simulink subsystem "Controller"  (R2025b)
settings: Solver=VariableStepAuto  StartTime=0.0  StopTime=10.0  RelTol=1e-3
libraries: slpidlib x1
settings Model: Creator=Admin  LastModifiedBy=Admin

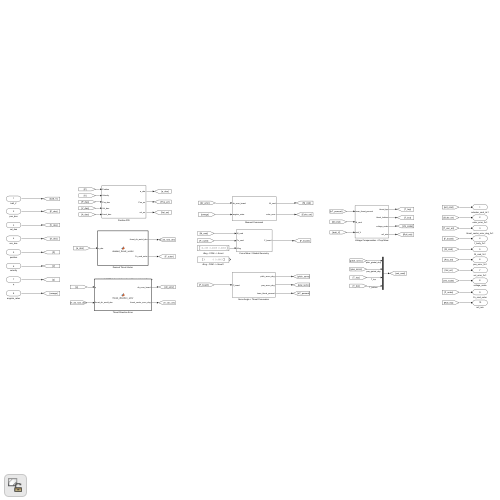
[thumbnail: Simulink's stored preview of the top-level diagram]
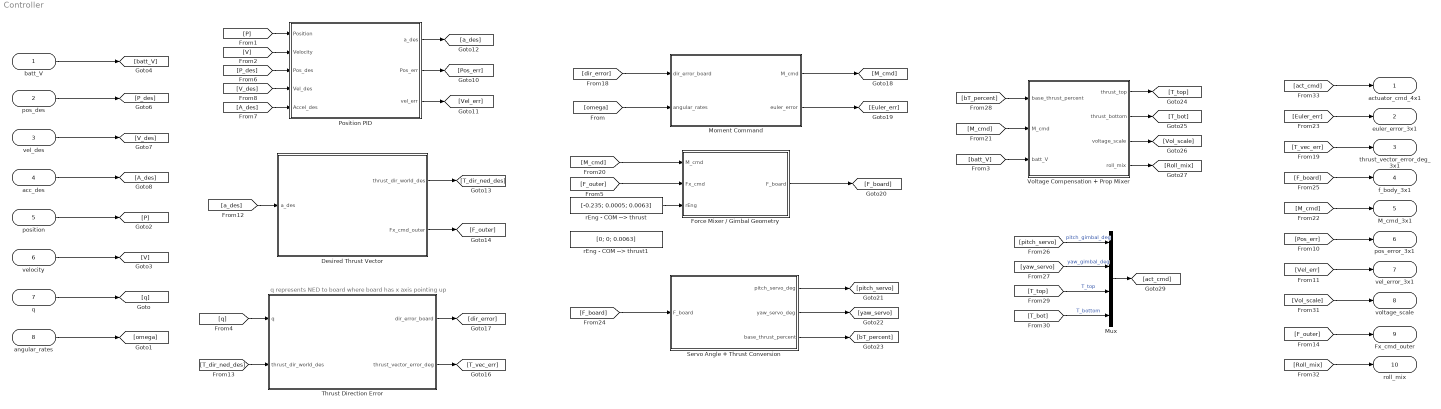
== system Controller ==
  note: q represents NED to board where board has x axis pointing up
  batt_V : Inport
  pos_des : Inport  Port=2
  vel_des : Inport  Port=3
  acc_des : Inport  Port=4
  position : Inport  Port=5
  velocity : Inport  Port=6
  q : Inport  Port=7
  angular_rates : Inport  Port=8
  Desired Thrust Vector : MATLAB Function  TreatAsAtomicUnit=on
  Force Mixer / Gimbal Geometry : Subsystem
  Moment Command : Subsystem
  Mux : Mux
  Position PID : Subsystem
  Servo Angle + Thrust Conversion : Subsystem
  Thrust Direction Error : MATLAB Function  TreatAsAtomicUnit=on
  Voltage Compensation + Prop Mixer : Subsystem
  rEng - COM --> thrust : Constant  Value=[-0.235; 0.0005; 0.0063]
  rEng - COM --> thrust1 : Constant  Value=[0; 0; 0.0063]
  actuator_cmd_4x1 : Outport
  euler_error_3x1 : Outport  Port=2
  thrust_vector_error_deg_3x1 : Outport  Port=3
  f_body_3x1 : Outport  Port=4
  M_cmd_3x1 : Outport  Port=5
  pos_error_3x1 : Outport  Port=6
  vel_error_3x1 : Outport  Port=7
  voltage_scale : Outport  Port=8
  Fx_cmd_outer : Outport  Port=9
  roll_mix : Outport  Port=10
  wires:
  [q] -> Thrust Direction Error/1(q)
  [omega] -> Moment Command/2(angular_rates)
  [P] -> Position PID/1(Position)
  [V] -> Position PID/2(Velocity)
  [P_des] -> Position PID/3(Pos_des)
  [A_des] -> Position PID/5(Accel_des)
  [V_des] -> Position PID/4(Vel_des)
  Position PID/2(Pos_err) -> [Pos_err]
  Position PID/3(vel_err) -> [Vel_err]
  [Pos_err] -> pos_error_3x1/1
  [Vel_err] -> vel_error_3x1/1
  [a_des] -> Desired Thrust Vector/1(a_des)
  Desired Thrust Vector/2(Fx_cmd_outer) -> [F_outer]
  [T_dir_ned_des] -> Thrust Direction Error/2(thrust_dir_world_des)
  [F_outer] -> Fx_cmd_outer/1
  [F_outer] -> Force Mixer / Gimbal Geometry/2(Fx_cmd)
  Thrust Direction Error/1(dir_error_board) -> [dir_error]
  Thrust Direction Error/2(thrust_vector_error_deg) -> [T_vec_err]
  [dir_error] -> Moment Command/1(dir_error_board)
  [T_vec_err] -> thrust_vector_error_deg_3x1/1
  Moment Command/1(M_cmd) -> [M_cmd]
  [M_cmd] -> Force Mixer / Gimbal Geometry/1(M_cmd)
  [M_cmd] -> M_cmd_3x1/1
  Moment Command/2(euler_error) -> [Euler_err]
  [Euler_err] -> euler_error_3x1/1
  Force Mixer / Gimbal Geometry/1(F_board) -> [F_board]
  [F_board] -> f_body_3x1/1
  Servo Angle + Thrust Conversion/1(pitch_servo_deg) -> [pitch_servo]
  Servo Angle + Thrust Conversion/2(yaw_servo_deg) -> [yaw_servo]
  Servo Angle + Thrust Conversion/3(base_thrust_percent) -> [bT_percent]
  [pitch_servo] -> Mux/1  "pitch_gimbal_deg"
  [yaw_servo] -> Mux/2  "yaw_gimbal_deg"
  [T_top] -> Mux/3  "T_top"
  [T_bot] -> Mux/4  "T_bottom"
  [Vol_scale] -> voltage_scale/1
  [Roll_mix] -> roll_mix/1
  Mux/1 -> [act_cmd]
  [act_cmd] -> actuator_cmd_4x1/1
  [bT_percent] -> Voltage Compensation + Prop Mixer/1(base_thrust_percent)
  [M_cmd] -> Voltage Compensation + Prop Mixer/2(M_cmd)
  [batt_V] -> Voltage Compensation + Prop Mixer/3(batt_V)
  Voltage Compensation + Prop Mixer/1(thrust_top) -> [T_top]
  Voltage Compensation + Prop Mixer/2(thrust_bottom) -> [T_bot]
  Voltage Compensation + Prop Mixer/3(voltage_scale) -> [Vol_scale]
  Voltage Compensation + Prop Mixer/4(roll_mix) -> [Roll_mix]
  Position PID/1(a_des) -> [a_des]
  Desired Thrust Vector/1(thrust_dir_world_des) -> [T_dir_ned_des]
  [F_board] -> Servo Angle + Thrust Conversion/1(F_board)
  batt_V/1 -> [batt_V]
  pos_des/1 -> [P_des]
  vel_des/1 -> [V_des]
  acc_des/1 -> [A_des]
  position/1 -> [P]
  velocity/1 -> [V]
  q/1 -> [q]
  angular_rates/1 -> [omega]
  rEng - COM --> thrust/1 -> Force Mixer / Gimbal Geometry/3(rEng)

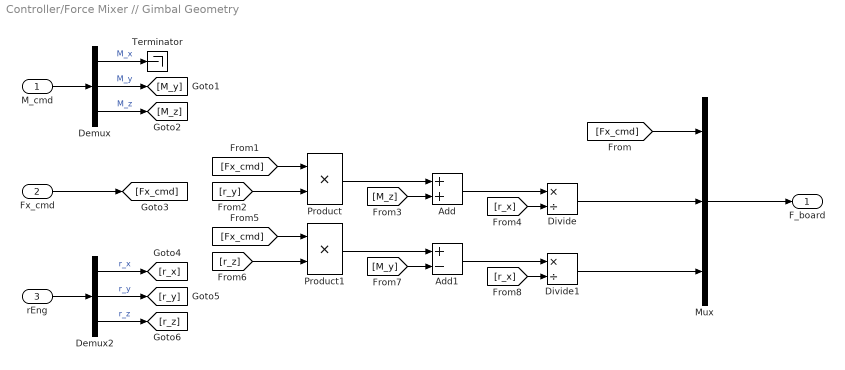
== system Controller/Force Mixer // Gimbal Geometry ==
  M_cmd : Inport
  Fx_cmd : Inport  Port=2
  rEng : Inport  Port=3
  Add : Sum
  Add1 : Sum  Inputs=+-
  Demux : Demux  Outputs=3
  Demux2 : Demux  Outputs=3
  Divide : Product  Inputs=*/
  Divide1 : Product  Inputs=*/
  Mux : Mux  Inputs=3
  Product : Product
  Product1 : Product
  Terminator : Terminator
  F_board : Outport
  wires:
  [r_z] -> Product1/2
  Product1/1 -> Add1/1
  Divide1/1 -> Mux/3
  Add1/1 -> Divide1/1
  [r_x] -> Divide1/2
  [Fx_cmd] -> Product1/1
  [M_y] -> Add1/2
  Divide/1 -> Mux/2
  [r_x] -> Divide/2
  [M_z] -> Add/2
  [r_y] -> Product/2
  [Fx_cmd] -> Product/1
  [Fx_cmd] -> Mux/1
  Demux2/1 -> [r_x]  "r_x"
  Demux2/3 -> [r_z]  "r_z"
  rEng/1 -> Demux2/1
  Demux2/2 -> [r_y]  "r_y"
  Fx_cmd/1 -> [Fx_cmd]
  Demux/3 -> [M_z]  "M_z"
  Demux/2 -> [M_y]  "M_y"
  Demux/1 -> Terminator/1  "M_x"
  Add/1 -> Divide/1
  Product/1 -> Add/1
  Mux/1 -> F_board/1
  M_cmd/1 -> Demux/1

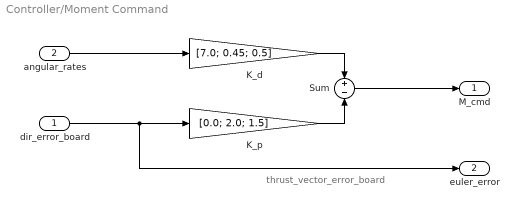
== system Controller/Moment Command ==
  note: thrust_vector_error_board
  dir_error_board : Inport
  angular_rates : Inport  Port=2
  K_d : Gain  Gain=[7.0; 0.45; 0.5]
  K_p : Gain  Gain=[0.0; 2.0; 1.5]
  Sum : Sum  Inputs=+-
  M_cmd : Outport
  euler_error : Outport  Port=2
  wires:
  Sum/1 -> M_cmd/1
  K_p/1 -> Sum/2
  K_d/1 -> Sum/1
  angular_rates/1 -> K_d/1
  dir_error_board/1 -> K_p/1, euler_error/1

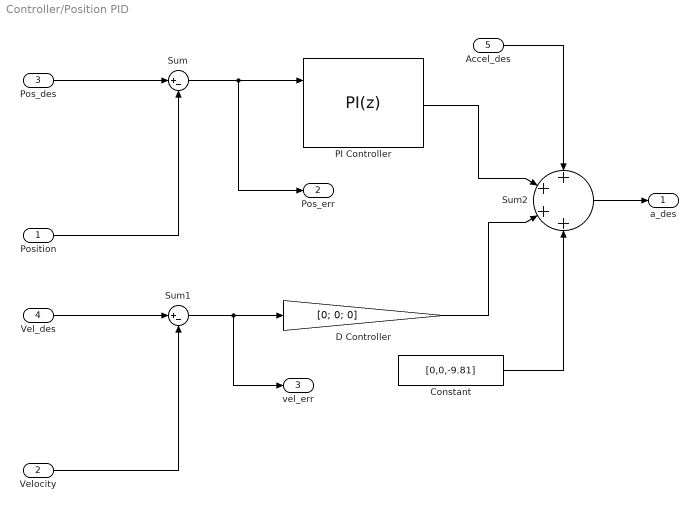
== system Controller/Position PID ==
  Position : Inport
  Velocity : Inport  Port=2
  Pos_des : Inport  Port=3
  Vel_des : Inport  Port=4
  Accel_des : Inport  Port=5
  Constant : Constant  Value=[0,0,-9.81]
  D Controller : Gain  Gain=[0; 0; 0]
  PI Controller : slpidlib/PID Controller  Controller=PI  Form=Parallel  TimeDomain=Discrete-time  UseExternalTs=off  SampleTime=-1  IntegratorMethod=Forward Euler  FilterMethod=Forward Euler  ControllerParametersSource=internal  P=-3*[0; 0; 0]  I=[0.0; 0.0; 0]  UseKiTs=on  D=0  UseExternalDerivativeSource=off  N=100  UseFilter=on  TunerSelectOption=Transfer Function Based (PID Tuner App)  InitialConditionSource=internal  InitialConditionForIntegrator=0  InitialConditionForFilter=0  DifferentiatorICPrevScaledInput=0  ExternalReset=level  TrackingMode=off  Kt=1  LimitOutput=off  SatLimitsSource=internal  UpperSaturationLimit=1  LowerSaturationLimit=-1  LinearizeAsGain=on  AntiWindupMode=clamping  Kb=1  LimitIntegrator=off  UpperIntegratorSaturationLimit=inf  LowerIntegratorSaturationLimit=-inf  RndMeth=Simplest  POutMin=[]  POutMax=[]  IOutMin=[]  IOutMax=[]  DOutMin=[]  DOutMax=[]  NOutMin=[]  NOutMax=[]  SumOutMin=[]  SumOutMax=[]  SaturationOutDataTypeStr=Inherit: Inherit via back propagation  SaturationOutMin=[]  SaturationOutMax=[]  PParamMin=[]  PParamMax=[]  IParamMin=[]  IParamMax=[]  DParamMin=[]  DParamMax=[]  NParamMin=[]  NParamMax=[]  KbParamMin=[]  KbParamMax=[]  KtParamMin=[]  KtParamMax=[]  KbOutMin=[]  KbOutMax=[]  KtOutMin=[]  KtOutMax=[]  IntegratorOutMin=[]  IntegratorOutMax=[]  FilterOutMin=[]  FilterOutMax=[]  SumI1OutMin=[]  SumI1OutMax=[]  SumI2OutMin=[]  SumI2OutMax=[]  SumI3OutMin=[]  SumI3OutMax=[]  SumI4OutMin=[]  SumI4OutMax=[]  SumDOutMin=[]  SumDOutMax=[]  DifferentiatorOutMin=[]  DifferentiatorOutMax=[]  FilterDiffOutCoefMin=[]  FilterDiffOutCoefMax=[]  ReciprocalOutMin=[]  ReciprocalOutMax=[]  SumDenOutMin=[]  SumDenOutMax=[]  SumNumOutMin=[]  SumNumOutMax=[]  DivideOutMin=[]  DivideOutMax=[]  UdiffTsProdOutMin=[]  UdiffTsProdOutMax=[]  NTsProdOutMin=[]  NTsProdOutMax=[]  UintegralTsProdOutMin=[]  UintegralTsProdOutMax=[]  UngainTsProdOutMin=[]  UngainTsProdOutMax=[]  ClampingZeroOutDataTypeStr=Inherit: Inherit via back propagation  ClampingZeroOutMin=[]  ClampingZeroOutMax=[]  FilterDenConstantOutDataTypeStr=Inherit: Inherit via back propagation  FilterDenConstantOutMin=[]  FilterDenConstantOutMax=[]  PCopyOutDataTypeStr=Inherit: Inherit via back propagation  PCopyOutMin=[]  PCopyOutMax=[]  NCopyOutDataTypeStr=Inherit: Inherit via back propagation  NCopyOutMin=[]  NCopyOutMax=[]  IntegratorContinuousStateAttributes=''  IntegratorStateMustResolveToSignalObject=off  IntegratorRTWStateStorageClass=Auto  FilterContinuousStateAttributes=''  FilterStateMustResolveToSignalObject=off  FilterRTWStateStorageClass=Auto  ParallelPVariant=InternalParameters  IdealPVariant=Disabled  IVariant=InternalParameters  DVariant=Disabled  IntegratorVariant=Discrete  SatVariant=Disabled  AWVariant=Passthrough  PCopyVariant=Disabled  TRVariant=Disabled  FdbkBlocksVariant=Forward  IdealPFdbkVariant=Disabled  SatFdbkVariant=Disabled  DerivativeFilterVariant=Disabled  NVariant=Disabled  NCopyVariant=Disabled_SignalSpec  FilterICVariant=Disabled  IntegratorICVariant=InternalICs  ExternalResetVariant=ExternalReset  TRSumVariant=Passthrough  SumFdbkVariant=Disabled  SumVariant=Sum_PI  TsampFilterVariant=InternalTs  TsampNgainVariant=Passthrough  TsampIntegralVariant=Disabled_SignalSpec  ExternalSaturationOutDataTypeStr=Inherit: Same as second input  DerivativeSourceVariant=Disabled  PreIntVariant=InternalPreInt
      settings: LibrarySourceBlock=mcbhdllib/Controls/Controllers/PI Controller
  Sum : Sum  Inputs=|+-
  Sum1 : Sum  Inputs=|+-
  Sum2 : Sum  Inputs=++++
  a_des : Outport
  Pos_err : Outport  Port=2
  vel_err : Outport  Port=3
  wires:
  Sum2/1 -> a_des/1
  Constant/1 -> Sum2/4
  D Controller/1 -> Sum2/3
  Accel_des/1 -> Sum2/1
  PI Controller/1 -> Sum2/2
  Sum/1 -> PI Controller/1, Pos_err/1
  Sum1/1 -> D Controller/1, vel_err/1
  Velocity/1 -> Sum1/2
  Vel_des/1 -> Sum1/1
  Position/1 -> Sum/2
  Pos_des/1 -> Sum/1

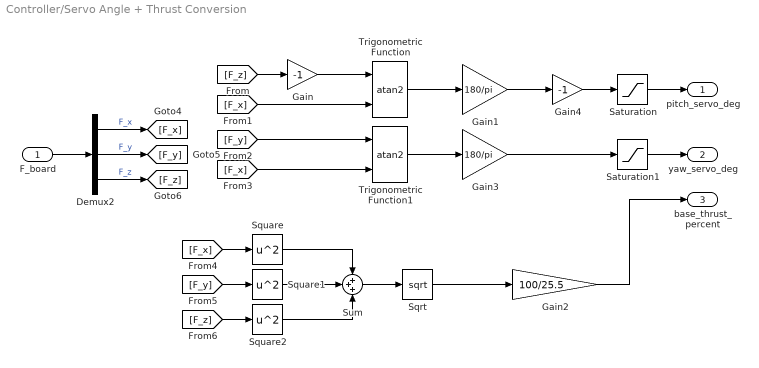
== system Controller/Servo Angle + Thrust Conversion ==
  F_board : Inport
  Demux2 : Demux  Outputs=3
  Gain : Gain  Gain=-1
  Gain1 : Gain  Gain=180/pi
  Gain2 : Gain  Gain=100/25.5
  Gain3 : Gain  Gain=180/pi
  Gain4 : Gain  Gain=-1
  Saturation : Saturate  UpperLimit=15  LowerLimit=-15
  Saturation1 : Saturate  UpperLimit=15  LowerLimit=-15
  Sqrt : Sqrt
  Square : Math  Operator=square
  Square1 : Math  Operator=square
  Square2 : Math  Operator=square
  Sum : Sum  Inputs=+++
  Trigonometric Function : Trigonometry  Operator=atan2  OutputSignalType=real
  Trigonometric Function1 : Trigonometry  Operator=atan2  OutputSignalType=real
  pitch_servo_deg : Outport
  yaw_servo_deg : Outport  Port=2
  base_thrust_percent : Outport  Port=3
  wires:
  Saturation1/1 -> yaw_servo_deg/1
  Saturation/1 -> pitch_servo_deg/1
  Gain4/1 -> Saturation/1
  Gain2/1 -> base_thrust_percent/1
  Sqrt/1 -> Gain2/1
  Sum/1 -> Sqrt/1
  Square2/1 -> Sum/3
  Square/1 -> Sum/1
  Square1/1 -> Sum/2
  [F_z] -> Square2/1
  [F_y] -> Square1/1
  [F_x] -> Square/1
  Gain3/1 -> Saturation1/1
  Gain1/1 -> Gain4/1
  [F_x] -> Trigonometric Function1/2
  [F_y] -> Trigonometric Function1/1
  Trigonometric Function1/1 -> Gain3/1
  Trigonometric Function/1 -> Gain1/1
  [F_x] -> Trigonometric Function/2
  Gain/1 -> Trigonometric Function/1
  [F_z] -> Gain/1
  Demux2/1 -> [F_x]  "F_x"
  F_board/1 -> Demux2/1
  Demux2/2 -> [F_y]  "F_y"
  Demux2/3 -> [F_z]  "F_z"

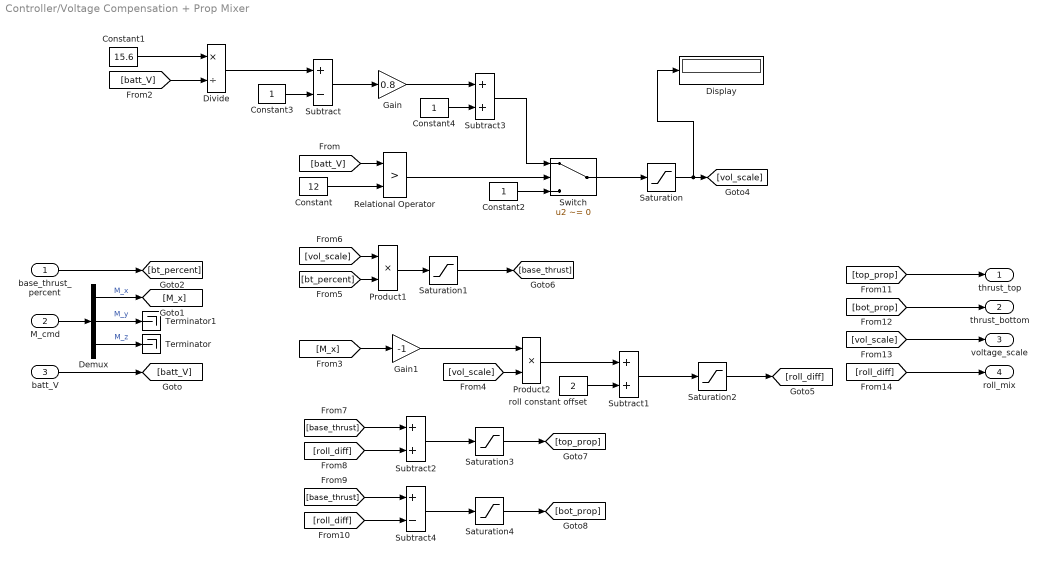
== system Controller/Voltage Compensation + Prop Mixer ==
  base_thrust_percent : Inport
  M_cmd : Inport  Port=2
  batt_V : Inport  Port=3
  Constant : Constant  Value=12
  Constant1 : Constant  Value=15.6
  Constant2 : Constant
  Constant3 : Constant
  Constant4 : Constant
  Demux : Demux  Outputs=3
  Display : Display
  Divide : Product  Inputs=*/
  Gain : Gain  Gain=0.8
  Gain1 : Gain  Gain=-1
  Product1 : Product
  Product2 : Product
  Relational Operator : RelationalOperator  Operator=>  OutDataTypeStr=boolean  RndMeth=Simplest  InputSameDT=off
  Saturation : Saturate  UpperLimit=1.07  LowerLimit=0.83
  Saturation1 : Saturate  UpperLimit=100  LowerLimit=0
  Saturation2 : Saturate  UpperLimit=8  LowerLimit=-8
  Saturation3 : Saturate  UpperLimit=100  LowerLimit=0
  Saturation4 : Saturate  UpperLimit=100  LowerLimit=0
  Subtract : Sum  Inputs=+-
  Subtract1 : Sum
  Subtract2 : Sum
  Subtract3 : Sum
  Subtract4 : Sum  Inputs=+-
  Switch : Switch  Criteria=u2 ~= 0  Threshold=12  SaturateOnIntegerOverflow=off  InputSameDT=off
  Terminator : Terminator
  Terminator1 : Terminator
  roll constant offset : Constant  Value=2
  thrust_top : Outport
  thrust_bottom : Outport  Port=2
  voltage_scale : Outport  Port=3
  roll_mix : Outport  Port=4
  wires:
  batt_V/1 -> [batt_V]
  Subtract/1 -> Gain/1
  base_thrust_percent/1 -> [bt_percent]
  M_cmd/1 -> Demux/1
  [vol_scale] -> Product1/1
  Constant4/1 -> Subtract3/2
  Saturation4/1 -> [bot_prop]
  Subtract4/1 -> Saturation4/1
  [roll_diff] -> Subtract4/2
  Saturation3/1 -> [top_prop]
  Constant2/1 -> Switch/3
  [batt_V] -> Divide/2
  [vol_scale] -> voltage_scale/1
  Gain/1 -> Subtract3/1
  Demux/1 -> [M_x]  "M_x"
  [M_x] -> Gain1/1
  Constant/1 -> Relational Operator/2
  Saturation1/1 -> [base_thrust]
  roll constant offset/1 -> Subtract1/2
  Switch/1 -> Saturation/1
  Constant1/1 -> Divide/1
  [base_thrust] -> Subtract2/1
  [vol_scale] -> Product2/2
  Subtract3/1 -> Switch/1
  Demux/2 -> Terminator1/1  "M_y"
  Relational Operator/1 -> Switch/2
  Saturation2/1 -> [roll_diff]
  Subtract1/1 -> Saturation2/1
  [batt_V] -> Relational Operator/1
  Product1/1 -> Saturation1/1
  [top_prop] -> thrust_top/1
  [base_thrust] -> Subtract4/1
  Constant3/1 -> Subtract/2
  Gain1/1 -> Product2/1
  Product2/1 -> Subtract1/1
  [roll_diff] -> roll_mix/1
  Subtract2/1 -> Saturation3/1
  [bot_prop] -> thrust_bottom/1
  Divide/1 -> Subtract/1
  Demux/3 -> Terminator/1  "M_z"
  [roll_diff] -> Subtract2/2
  [bt_percent] -> Product1/2
  Saturation/1 -> [vol_scale], Display/1

== matlab function Controller/Thrust Direction Error ==
  data: q input; dir_error_board output; thrust_dir_world_des input; thrust_vector_error_deg output
function [dir_error_board, thrust_vector_error_deg] = thrust_direction_error(q, thrust_dir_world_des)

RAD_TO_DEG = 180/pi;

q = q(:) / norm(q);

thrust_axis_board = [1;0;0];

% Current thrust direction in NED/world frame
thrust_dir_world = body2ned(thrust_axis_board, q);
thrust_dir_world = thrust_dir_world / norm(thrust_dir_world);

% Normalize desired direction
thrust_dir_world_des = thrust_dir_world_des(:);
thrust_dir_world_des = thrust_dir_world_des / norm(thrust_dir_world_des);

% Error axis in world frame
e_world = cross(thrust_dir_world, thrust_dir_world_des); % Which way do 

% Rotate into body frame
dir_error_board = ned2body(e_world, q);

desired_board = ned2body(thrust_dir_world_des, q);

total_error_rad = asin(min(max(norm(e_world),0),1));

pitch_error_rad = atan2(desired_board(3), desired_board(1)); % Meant to be error, not desired. Des kind of represents the error correction if you really think about it FOR HOVER. Used for telemetry anyways 
yaw_error_rad   = atan2(desired_board(2), desired_board(1)); % Meant to be error, not desired. Des kind of represents the error correction if you really think about it FOR HOVER. Used for telemetry anyways

thrust_vector_error_deg = [
    total_error_rad;
    pitch_error_rad;
    yaw_error_rad
] * RAD_TO_DEG;

% No roll control about thrust axis
dir_error_board(1) = 0;

== matlab function Controller/Desired Thrust Vector ==
  data: a_des input; thrust_dir_world_des output; Fx_cmd_outer output
function [thrust_dir_world_des, Fx_cmd_outer] = desired_thrust_vector(a_des)

mass = 1.42; % kg
MAX_THRUST_N = 30; % Newtons

F_des_world = mass * a_des;
F_mag = norm(F_des_world);

if F_mag < 1e-3
    thrust_dir_world_des = [0;0;-1];
    Fx_cmd_outer = 0;
else
    thrust_dir_world_des = F_des_world / F_mag;
    Fx_cmd_outer = min(max(F_mag, 0), MAX_THRUST_N);
end
